simulink model "Controlador_LQR_implementation"  (R2026a)
settings: Solver=FixedStepDiscrete  StopTime=inf  FixedStep=Ts  EnableMultiTasking=on
InitFcn:
  | init_BOOT
values from neighbouring files (symbols this model uses):
  AW_activo = true    [init_BOOT.m]
  DeltaD_max = single(DeltaD_max)    [init_BOOT.m]
  DeltaD_min = single(DeltaD_min)    [init_BOOT.m]
  Ki_LQR = K_LQR(3)    [init_BOOT.m]
  Ku_LQR = K_LQR(2)    [init_BOOT.m]
  Kx_LQR = K_LQR(1)    [init_BOOT.m]
  Ts = 250e-6    (= 0.00025)    [init_BOOT.m]
undefined symbols (not defined in the file or in its folder): DiscIntNeverNeededParam
settings Model: SILPILModeSetting=veronly  ExtModeTrigDuration=2  Creator=Usuario  LastModifiedBy=pablo_elizondo17
settings HardwareCC: ProdBitPerInt=16.0  ProdBitPerPointer=16.0  ProdBitPerSizeT=16.0  ProdBitPerPtrDiffT=16.0  ProdWordSize=8.0  ProdHWDeviceType=Atmel->AVR
settings ModelReferenceCC: PropagateVarSize=During execution
settings RTWCC: SystemTargetFile=ert.tlc  HardwareBoard=Arduino Mega 2560  TLCOptions=-aInlineSetEventsForThisBaseRateFcn=TLC_FALSE -aSuppressMultiTaskScheduler=TLC_FALSE -aRateBasedStepFcn=1  Toolchain=Arduino AVR  BuildConfiguration=Faster Runs  Description=Embedded Coder
settings ERTTargetCC: ExtModeTransport=1.0  ExtModeAutomaticAllocSize=off  ExtModeStaticAllocSize=2048.0  RootIOFormat=Structure reference  CodeInterfacePackaging=Reusable function  SupportContinuousTime=on  SupportVariableSizeSignals=on

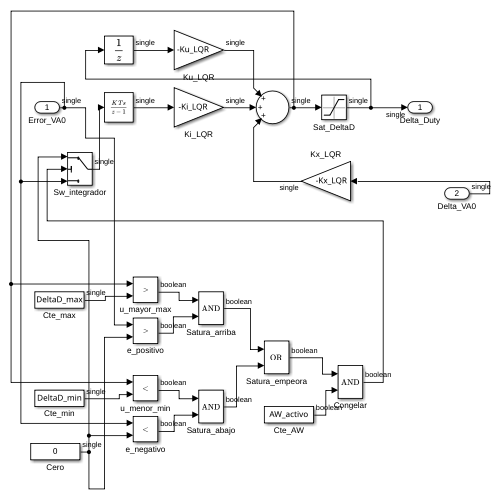
[thumbnail: Simulink's stored preview of the top-level diagram]
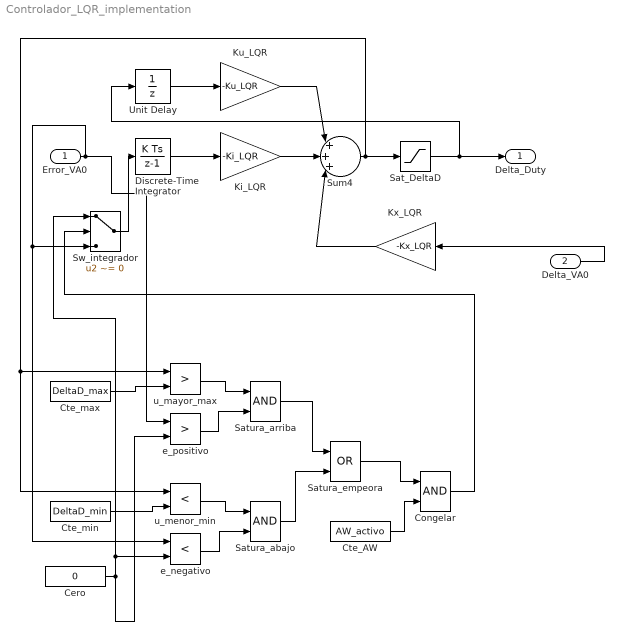
== system Controlador_LQR_implementation ==
  Error_VA0 : Inport  OutDataTypeStr=single  PortDimensions=1  SampleTime=[0.00025000000000000001,0]
  Delta_VA0 : Inport  Port=2  OutDataTypeStr=single  PortDimensions=1  SampleTime=[0.00025000000000000001,0]
  Cero : Constant  Value=0  OutDataTypeStr=single
  Congelar : Logic  AllPortsSameDT=off  OutDataTypeStr=boolean
  Cte_AW : Constant  Value=AW_activo  OutDataTypeStr=boolean
  Cte_max : Constant  Value=DeltaD_max  OutDataTypeStr=single
  Cte_min : Constant  Value=DeltaD_min  OutDataTypeStr=single
  Discrete-Time Integrator : DiscreteIntegrator  SampleTime=Ts  OutDataTypeStr=single  ICPrevOutput=DiscIntNeverNeededParam  ICPrevScaledInput=DiscIntNeverNeededParam
  Ki_LQR : Gain  Gain=-Ki_LQR  OutDataTypeStr=Inherit: Same as input  ParamDataTypeStr=Inherit: Same as input
  Ku_LQR : Gain  Gain=-Ku_LQR  OutDataTypeStr=Inherit: Same as input  ParamDataTypeStr=Inherit: Same as input
  Kx_LQR : Gain  Gain=-Kx_LQR  OutDataTypeStr=Inherit: Same as input  ParamDataTypeStr=Inherit: Same as input
  Sat_DeltaD : Saturate  UpperLimit=DeltaD_max  LowerLimit=DeltaD_min
  Satura_abajo : Logic  AllPortsSameDT=off  OutDataTypeStr=boolean
  Satura_arriba : Logic  AllPortsSameDT=off  OutDataTypeStr=boolean
  Satura_empeora : Logic  Operator=OR  AllPortsSameDT=off  OutDataTypeStr=boolean
  Sum4 : Sum  Inputs=|+++|  OutDataTypeStr=single
  Sw_integrador : Switch  Criteria=u2 ~= 0  SaturateOnIntegerOverflow=off  InputSameDT=off
  Unit Delay : UnitDelay  SampleTime=Ts
  e_negativo : RelationalOperator  Operator=<  OutDataTypeStr=boolean  RndMeth=Simplest  InputSameDT=off
  e_positivo : RelationalOperator  Operator=>  OutDataTypeStr=boolean  RndMeth=Simplest  InputSameDT=off
  u_mayor_max : RelationalOperator  Operator=>  OutDataTypeStr=boolean  RndMeth=Simplest  InputSameDT=off
  u_menor_min : RelationalOperator  Operator=<  OutDataTypeStr=boolean  RndMeth=Simplest  InputSameDT=off
  Delta_Duty : Outport  OutDataTypeStr=single  PortDimensions=1  SampleTime=[0.00025000000000000001,0]
  wires:
  Unit Delay/1 -> Ku_LQR/1
  Discrete-Time Integrator/1 -> Ki_LQR/1
  Delta_VA0/1 -> Kx_LQR/1
  Ku_LQR/1 -> Sum4/1
  Ki_LQR/1 -> Sum4/2
  Kx_LQR/1 -> Sum4/3
  Sum4/1 -> u_mayor_max/1, u_menor_min/1, Sat_DeltaD/1
  Sat_DeltaD/1 -> Unit Delay/1, Delta_Duty/1
  Cte_max/1 -> u_mayor_max/2
  Error_VA0/1 -> e_negativo/1, Sw_integrador/3, e_positivo/1
  Cero/1 -> e_positivo/2, e_negativo/2, Sw_integrador/1
  Cte_min/1 -> u_menor_min/2
  u_mayor_max/1 -> Satura_arriba/1
  e_positivo/1 -> Satura_arriba/2
  u_menor_min/1 -> Satura_abajo/1
  e_negativo/1 -> Satura_abajo/2
  Satura_arriba/1 -> Satura_empeora/1
  Satura_abajo/1 -> Satura_empeora/2
  Satura_empeora/1 -> Congelar/1
  Cte_AW/1 -> Congelar/2
  Congelar/1 -> Sw_integrador/2
  Sw_integrador/1 -> Discrete-Time Integrator/1
